simulink library "sm_wheel_loader_lib"  (R2025a)
settings: Solver=VariableStepAuto  StartTime=0.0  StopTime=10.0  RelTol=1e-3
undefined symbols (not defined in the file): AToTOrificeVector, BiPOrificeVector, boomHEArea, boomREArea, BToTOrificeVector, fluids, GRake, GToothL, GToothR, HMPST, HydFcnParams, logLoad, Position, PToAOrificeVector, PToBOrificeVector, RakeL, RakeR, testInput, Wheel_Loader, X, Y, Z
libraries: sm_lib x694, fl_lib x183, nesl_utility x74, SimscapeFluids_lib x62, sdl_lib x25, cvt_components_lib x25, simulink_extras x5, $bdroot x4, wheel_loader_contact_lib x4, ee_lib x2, SignalEditorBlockLib x1, batteryecm_lib x1
(part 3 of 26)

== system sm_wheel_loader_lib/CVT Power Split Hydromechanical/HRB ==
  str : Inport
  Constant : Constant  Value=HMPST.HRB.Pump.effVol
  Constant1 : Constant  Value=HMPST.HRB.Pump.effMech
  Custom Hydraulic Fluid : fl_lib/Isothermal Liquid/Utilities/Isothermal Liquid Properties (IL)  rho_L_atm=850 kg/m^3  bulk_modulus_model=foundation.enum.bulk_modulus_model.const  beta_gain=6  beta_L_atm=0.8e9 Pa  nu_atm=18e-6 m^2/s  p_atm=0.101325 MPa  p_min=1 Pa  properties_range_check=simscape.enum.assert.action.error  air_fraction=0.005  polytropic_index=1.0  rho_g_atm=1.225 kg/m^3  air_dissolution_model=simscape.enum.onoff.off  p_crit=3 MPa
      settings: LibrarySourceBlock=|
      | fl_lib/Hydraulic/Hydraulic Utilities/Custom Hydraulic
      | Fluid
  Gas-Charged Accumulator : SimscapeFluids_lib/Isothermal Liquid/Tanks & Accumulators/Gas-Charged Accumulator (IL)  capacity=HMPST.HRB.Accumulator.volTotal m^3  dead_volume=HMPST.HRB.Accumulator.volGasMin m^3  p_precharge=HMPST.HRB.Accumulator.pPrecharge MPa  k_sh=1.4  stiff_coeff=1e10 Pa/m^3  dynamic_compressibility=simscape.enum.onoff.off  liquid_volume_specify=on  liquid_volume_priority=High  liquid_volume=HMPST.HRB.Accumulator.volLiquidInit m^3  liquid_volume_nominal_specify=off  liquid_volume_nominal_value=1  liquid_volume_nominal_unit=m^3  liquid_mass_specify=off  liquid_mass_priority=None  liquid_mass=5 kg  liquid_mass_nominal_specify=off  liquid_mass_nominal_value=1  liquid_mass_nominal_unit=kg  p_I_specify=on  p_I_priority=None  p_I=HMPST.HRB.Accumulator.pLiquidInit Pa  p_I_nominal_specify=off  p_I_nominal_value=1  p_I_nominal_unit=Pa
      settings: InternalSimscapePortConfiguration="{\"Bottom\":[],\"Left\":[],\"Right\":[{\"id\":\"A\",\"label\":\"A\",\"type\":\"foundation.isothermal_liquid.isothermal_liquid\"}],\"Top\":[]}"
      settings: LibrarySourceBlock=|
      | sh_lib/Accumulators/Gas-Charged
      | Accumulator
  Maximum displacement : fl_lib/Physical Signals/Nonlinear Operators/PS Saturation  upper_limit=HMPST.HRB.Pump.dispMax m^3/rad  lower_limit=HMPST.HRB.Pump.dispMin m^3/rad  ZeroCross=true
  Mechanical Rotational Reference : fl_lib/Mechanical/Rotational Elements/Mechanical Rotational Reference
  Pressure Relief Valve : SimscapeFluids_lib/Isothermal Liquid/Valves & Orifices/Pressure Control Valves/Pressure Relief Valve (IL)  set_pressure_spec=foundation.enum.constant_controlled.constant  opening_spec=1  pressure_spec=fluids.isothermal_liquid.valves_orifices.enum.pressure_control_spec.dp  p_set_gauge=0.1 MPa  p_set_differential=HMPST.HRB.PRV.pDiffOpen bar  p_range=HMPST.HRB.PRV.pRange bar  area_max=HMPST.HRB.PRV.aMax m^2  area_leak=HMPST.HRB.PRV.aLeak m^2  p_diff_TLU=[30.15e5 : 15e3 : 31.35e5] Pa  p_gauge_TLU=[0.2 : 0.2 : 1.2] MPa  valve_area_TLU=[1 : 1 : 9] .* 1e-5 m^2  vol_flow_TLU=[1e-09, 3.6e-05, 8.9e-05, .00015, .00023, .00031] m^3/s  area=inf m^2  Cd=0.7  Re_c=12  smoothing_factor=0  pressure_recovery=false  opening_dynamics=1  tau=HMPST.HRB.PRV.tsOpen s
      settings: InternalSimscapePortConfiguration="{\"Bottom\":[],\"Left\":[{\"id\":\"A\",\"label\":\"A\",\"type\":\"foundation.isothermal_liquid.isothermal_liquid\"}],\"Right\":[{\"id\":\"B\",\"label\":\"B\",\"type\":\"foundation.isothermal_liquid.isothermal_liquid\"}],\"Top\":[]}"
      settings: LibrarySourceBlock=|
      | sh_lib/Valves/Pressure Control
      | Valves/Pressure Relief
      | Valve
  Reservoir : fl_lib/Isothermal Liquid/Elements/Reservoir (IL)  reservoir_type=foundation.enum.constant_controlled.constant  pressure_spec=foundation.enum.pressure_spec.atmospheric  reservoir_pressure=0.101325 MPa
      settings: LibrarySourceBlock=fl_lib/Hydraulic/Hydraulic Elements/Hydraulic Reference
  Simulink-PS Converter : nesl_utility/Simulink-PS Converter  PhysicalDomain=network_engine_domain  SubClassName=ps_input  LeftPortType=input  RightPortType=output  PseudoPeriodic=off  Frequencies=[]  NoiseDistribution=none  NoiseParameters=[]  Unit=1  AffineConversion=off  FilteringAndDerivatives=zero  SimscapeFilterOrder=1  InputFilterTimeConstant=0.001  UdotUserProvided=1
  Simulink-PS Converter1 : nesl_utility/Simulink-PS Converter  PhysicalDomain=network_engine_domain  SubClassName=ps_input  LeftPortType=input  RightPortType=output  PseudoPeriodic=off  Frequencies=[]  NoiseDistribution=none  NoiseParameters=[]  Unit=1  AffineConversion=off  FilteringAndDerivatives=zero  SimscapeFilterOrder=1  InputFilterTimeConstant=0.001  UdotUserProvided=1
  Simulink-PS Converter3 : nesl_utility/Simulink-PS Converter  PhysicalDomain=network_engine_domain  SubClassName=ps_input  LeftPortType=input  RightPortType=output  PseudoPeriodic=off  Frequencies=[]  NoiseDistribution=none  NoiseParameters=[]  Unit=m  AffineConversion=off  FilteringAndDerivatives=zero  SimscapeFilterOrder=1  InputFilterTimeConstant=0.001  UdotUserProvided=1
  Subsystem : Subsystem
  Transfer Fcn7 : TransferFcn  Numerator=HMPST.Ctrl.HRB.Num  Denominator=HMPST.Ctrl.HRB.Den
  Variable-Displacement Hydraulic Machine : SimscapeFluids_lib/Isothermal Liquid/Pumps & Motors/Variable-Displacement Motor (IL)  leakage_friction_spec=fluids.isothermal_liquid.pumps_motors.enum.pump_motor_loss_spec.input_efficiency  displacement_nominal=30 cm^3/rev  omega_nominal=1800 rpm  p_nominal=10 MPa  vol_eff_nominal=0.92  mech_eff_nominal=0.88  no_load_torque=0 N*m  p_diff_eff_TLU=[.1, 1, 2] MPa  omega_eff_TLU=[250, 500, 1000, 2000, 3000, 4000] rpm  displacement_eff_TLU=[-30, -19, 19, 30] cm^3/rev  vol_eff_TLU=repmat([.816, .908, .954, .977, .981, .984; .325, .663, .831, .916, .925, .946; .137, .568, .78, .892, .893, .91], 1, 1, 4)  mech_eff_TLU=repmat([.996, .996, .996, .996, .996, .996; .988, .989, .989, .989, .989, .99; .981, .981, .982, .982, .983, .984], 1, 1, 4)  p_diff_loss_TLU=[.1, 1, 2] MPa  omega_loss_TLU=[250, 500, 1000, 2000, 3000, 4000] rpm  displacement_loss_TLU=[-30, -19, 19, 30] cm^3/rev  vol_loss_TLU=repmat(1e-3 * [.023, .023, .023, .023, .0285, .032; .0844, .0842, .0845, .084, .1125, .108; .1079, .108, .11, .108, .1605, .18], 1, 1, 4) m^3/s  mech_loss_TLU=repmat([.002, .002, .002, .002, .002, .002; .0607, .0556, .0556, .0556, .0556, .0505; .1937, .1937, .1833, .1833, .1729, .1626], 1, 1, 4) N*m  vol_eff_min=1e-3  vol_eff_max=1  mech_eff_min=1e-3  mech_eff_max=1  pressure_threshold=1e-3 MPa  omega_threshold=100 rpm  displacement_threshold=0.1 cm^3/rev  supplied_range_check=simscape.enum.assert.action.none  motor_mode_check=simscape.enum.assert.action.none  pressure_check=simscape.enum.assert.action.none  p_min_valid=0.101325 MPa
      settings: InternalSimscapePortConfiguration="{\"Bottom\":[{\"id\":\"B\",\"label\":\"B\",\"type\":\"foundation.isothermal_liquid.isothermal_liquid\"}],\"Left\":[{\"id\":\"D\",\"label\":\"D\",\"type\":\"input\"},{\"id\":\"EV\",\"label\":\"EV\",\"type\":\"input\"},{\"id\":\"EM\",\"label\":\"EM\",\"type\":\"input\"}],\"Right\":[{\"id\":\"R\",\"label\":\"R\",\"type\":\"foundation.mechanical.rotational.rotational\"},{\"id\":\"C\",\"label\":\"C\",\"type\":\"foundation.mechanical.rotational.rotational\"}],\"Top\":[{\"id\":\"A\",\"label\":\"A\",\"type\":\"foundation.isothermal_liquid.isothermal_liquid\"}]}"
      settings: LibrarySourceBlock=|
      | sh_legacy_lib/Hydraulic Machines/Variable-Displacement
      | Hydraulic Machine
      | (External
      | Efficiencies)
  stroke2disp : fl_lib/Physical Signals/Functions/PS Gain  gain=HMPST.HRB.Pump.stroke2disp m^2/rad
  R : PMIOPort  Side=Right
  p : Outport
  wires:
  Transfer Fcn7/1 -> Simulink-PS Converter3/1  "HRB"
  str/1 -> Transfer Fcn7/1
  Constant/1 -> Simulink-PS Converter/1
  Constant1/1 -> Simulink-PS Converter1/1
  Subsystem/1(p) -> p/1  "P_acc (MPa)"
  connections:
  Subsystem/LConn1 -- Pressure Relief Valve/LConn1 -- Variable-Displacement Hydraulic Machine/RConn3 -- Gas-Charged Accumulator/RConn1
  stroke2disp/RConn1 -- Maximum displacement/LConn1
  R/RConn1 -- Variable-Displacement Hydraulic Machine/RConn1
  Simulink-PS Converter3/RConn1 -- stroke2disp/LConn1
  Maximum displacement/RConn1 -- Variable-Displacement Hydraulic Machine/LConn1
  Pressure Relief Valve/RConn1 -- Reservoir/LConn1 -- Variable-Displacement Hydraulic Machine/LConn4 -- Custom Hydraulic Fluid/RConn1
  Mechanical Rotational Reference/LConn1 -- Variable-Displacement Hydraulic Machine/RConn2
  Variable-Displacement Hydraulic Machine/LConn3 -- Simulink-PS Converter1/RConn1
  Variable-Displacement Hydraulic Machine/LConn2 -- Simulink-PS Converter/RConn1

== system sm_wheel_loader_lib/CVT Power Split Hydromechanical/Hydrostatic ==
  Ctrl : Inport
  CV Charge Pump : fl_lib/Isothermal Liquid/Elements/Constant Volume Chamber (IL)  volume=1e-4 m^3  p_I_specify=off  p_I_priority=High  p_I=0.101325 MPa  p_I_nominal_specify=off  p_I_nominal_value=1  p_I_nominal_unit=MPa
      settings: InternalSimscapePortConfiguration="{\"Bottom\":[],\"Left\":[{\"id\":\"A\",\"label\":\"A\",\"type\":\"foundation.isothermal_liquid.isothermal_liquid\"}],\"Right\":[],\"Top\":[]}"
  CV Motor A : fl_lib/Isothermal Liquid/Elements/Constant Volume Chamber (IL)  volume=1e-4 m^3  p_I_specify=off  p_I_priority=High  p_I=0.101325 MPa  p_I_nominal_specify=off  p_I_nominal_value=1  p_I_nominal_unit=MPa
      settings: InternalSimscapePortConfiguration="{\"Bottom\":[],\"Left\":[{\"id\":\"A\",\"label\":\"A\",\"type\":\"foundation.isothermal_liquid.isothermal_liquid\"}],\"Right\":[],\"Top\":[]}"
  CV Motor B : fl_lib/Isothermal Liquid/Elements/Constant Volume Chamber (IL)  volume=1e-4 m^3  p_I_specify=off  p_I_priority=High  p_I=0.101325 MPa  p_I_nominal_specify=off  p_I_nominal_value=1  p_I_nominal_unit=MPa
      settings: InternalSimscapePortConfiguration="{\"Bottom\":[],\"Left\":[{\"id\":\"A\",\"label\":\"A\",\"type\":\"foundation.isothermal_liquid.isothermal_liquid\"}],\"Right\":[],\"Top\":[]}"
  CV Pump A : fl_lib/Isothermal Liquid/Elements/Constant Volume Chamber (IL)  volume=1e-4 m^3  p_I_specify=off  p_I_priority=High  p_I=0.101325 MPa  p_I_nominal_specify=off  p_I_nominal_value=1  p_I_nominal_unit=MPa
      settings: InternalSimscapePortConfiguration="{\"Bottom\":[],\"Left\":[{\"id\":\"A\",\"label\":\"A\",\"type\":\"foundation.isothermal_liquid.isothermal_liquid\"}],\"Right\":[],\"Top\":[]}"
  CV Pump B : fl_lib/Isothermal Liquid/Elements/Constant Volume Chamber (IL)  volume=1e-4 m^3  p_I_specify=off  p_I_priority=High  p_I=0.101325 MPa  p_I_nominal_specify=off  p_I_nominal_value=1  p_I_nominal_unit=MPa
      settings: InternalSimscapePortConfiguration="{\"Bottom\":[],\"Left\":[{\"id\":\"A\",\"label\":\"A\",\"type\":\"foundation.isothermal_liquid.isothermal_liquid\"}],\"Right\":[],\"Top\":[]}"
  Charge Pump : Subsystem  Tag=PublishSubsystem  mask{chgPumpNomDisp=chgPumpNomDisp, chgPumpNomSpd=chgPumpNomSpd, chgPumpNomPressGain=chgPumpNomPressGain, chgPumpNomVolEff=chgPumpNomVolEff, chgPumpNomMechEff=chgPumpNomMechEff, chgPumpChkvPdiff=chgPumpChkvPdiff, chgPumpChkvPrange=chgPumpChkvPrange, chgPumpChkvAmax=chgPumpChkvAmax, chgPumpChkvAleak=chgPumpChkvAleak}
      mask prompts: chgPumpNomDisp "Displacement (cm^3/rev)"; chgPumpNomSpd "Nominal Angular Velocity (rpm)"; chgPumpNomPressGain "Nominal pressure gain (MPa)"; chgPumpNomVolEff "Nominal Volumetric Efficiency (0-1)"; chgPumpNomMechEff "Nominal Mechanical Efficiency (0-1)"; chgPumpChkvPdiff "Set pressure differential (MPa)"; chgPumpChkvPrange "Pressure regulation range (MPa)"; chgPumpChkvAmax "Maximum opening area (m^2)"; chgPumpChkvAleak "Leakage area (m^2)"
      mask TypeOptions chgPumpNomDisp: Pump/displacement
      mask TypeOptions chgPumpNomSpd: Pump/omega_nominal
      mask TypeOptions chgPumpNomPressGain: Pump/p_nominal
      mask TypeOptions chgPumpNomVolEff: Pump/vol_eff_nominal
      mask TypeOptions chgPumpNomMechEff: Pump/mech_eff_nominal
      mask TypeOptions chgPumpChkvPdiff:
      | Pressure
      | Relief
      | Valve/p_set_differential
      mask TypeOptions chgPumpChkvPrange:
      | Pressure
      | Relief
      | Valve/p_range
      mask TypeOptions chgPumpChkvAmax:
      | Pressure
      | Relief
      | Valve/area_max
      mask TypeOptions chgPumpChkvAleak:
      | Pressure
      | Relief
      | Valve/area_leak
      mask DialogControl grp_chg_pump Prompt: Pump
      mask DialogControl grp_chg_pump_prv Prompt: Pressure Relief Valve
      mask Display:
      | % Circle
      | color('green')
      | plot(2*cos(linspace(0, 2*pi, 100)), 2*sin(linspace(0, 2*pi, 100)))
      | % Triangle
      | patch([1 0.4 0.4]*2, [0,-0.4,0.4]*2,[45 48 173]/255)
      | % Boundary
      | color('white')
      | plot(-2, -2)
      | plot(2, 2)
  Check Valve A : SimscapeFluids_lib/Isothermal Liquid/Valves & Orifices/Directional Control Valves/Check Valve (IL)  opening_spec=2*(fluids.isothermal_liquid.valves_orifices.enum.PressureOpeningSpec.Linear)-1  pressure_control_spec=fluids.isothermal_liquid.valves_orifices.enum.pressure_control_spec.dp  p_crack_differential=p_crack_differential MPa  p_crack_gauge=0.1 MPa  press_max_differential=press_max_differential MPa  press_max_gauge=0.2 MPa  area_max=chkv_area_max m^2  area_leak=chkv_area_leak m^2  p_diff_TLU=[0.01 : 0.01 : 0.1] MPa  valve_area_TLU=[1e-10, 1e-05, 2e-05, 3e-05, 4e-05, 5e-05, 6e-05, 7.5e-05, 8.5e-05, .0001] m^2  vol_flow_TLU=[.000358, .045, .11, .191, .284, .39, .505, .63, .764, .905] .* 1e-3 m^3/s  area=inf m^2  Cd=0.64  Re_c=150  smoothing_factor=0.01  pressure_recovery=simscape.enum.onoff.off  opening_dynamics=simscape.enum.onoff.off  tau=0.1 s
      settings: InternalSimscapePortConfiguration="{\"Bottom\":[],\"Left\":[{\"id\":\"A\",\"label\":\"A\",\"type\":\"foundation.isothermal_liquid.isothermal_liquid\"}],\"Right\":[{\"id\":\"B\",\"label\":\"B\",\"type\":\"foundation.isothermal_liquid.isothermal_liquid\"}],\"Top\":[]}"
  Check Valve B : SimscapeFluids_lib/Isothermal Liquid/Valves & Orifices/Directional Control Valves/Check Valve (IL)  opening_spec=2*(fluids.isothermal_liquid.valves_orifices.enum.PressureOpeningSpec.Linear)-1  pressure_control_spec=fluids.isothermal_liquid.valves_orifices.enum.pressure_control_spec.dp  p_crack_differential=p_crack_differential MPa  p_crack_gauge=0.1 MPa  press_max_differential=press_max_differential MPa  press_max_gauge=0.2 MPa  area_max=chkv_area_max m^2  area_leak=chkv_area_leak m^2  p_diff_TLU=[0.01 : 0.01 : 0.1] MPa  valve_area_TLU=[1e-10, 1e-05, 2e-05, 3e-05, 4e-05, 5e-05, 6e-05, 7.5e-05, 8.5e-05, .0001] m^2  vol_flow_TLU=[.000358, .045, .11, .191, .284, .39, .505, .63, .764, .905] .* 1e-3 m^3/s  area=inf m^2  Cd=0.64  Re_c=150  smoothing_factor=0.01  pressure_recovery=simscape.enum.onoff.off  opening_dynamics=simscape.enum.onoff.off  tau=0.1 s
      settings: InternalSimscapePortConfiguration="{\"Bottom\":[],\"Left\":[{\"id\":\"A\",\"label\":\"A\",\"type\":\"foundation.isothermal_liquid.isothermal_liquid\"}],\"Right\":[{\"id\":\"B\",\"label\":\"B\",\"type\":\"foundation.isothermal_liquid.isothermal_liquid\"}],\"Top\":[]}"
  Gain1 : Gain  Gain=pumpNomDisp
  Gain2 : Gain  Gain=-1
  Mechanical Rotational Reference : fl_lib/Mechanical/Rotational Elements/Mechanical Rotational Reference
  Mechanical Rotational Reference1 : fl_lib/Mechanical/Rotational Elements/Mechanical Rotational Reference
  Motor : SimscapeFluids_lib/Isothermal Liquid/Pumps & Motors/Fixed-Displacement Motor (IL)  leakage_friction_spec=fluids.isothermal_liquid.pumps_motors.enum.MotorLossSpec.Analytical  displacement=motorNomDisp cm^3/rev  omega_nominal=motorNomSpd rpm  p_nominal=motorNomPressDrop MPa  vol_eff_nominal=motorNomVolEff  mech_eff_nominal=motorNomMechEff  no_load_torque=0 N*m  p_diff_eff_TLU=[.1, 1, 2] MPa  omega_eff_TLU=[25, 50, 100, 200, 300, 400] rad/s  vol_eff_TLU=[.816, .908, .954, .977, .981, .984; .325, .663, .831, .916, .925, .946; .137, .568, .78, .892, .893, .91]  mech_eff_TLU=[.996, .996, .996, .996, .996, .996; .988, .989, .989, .989, .989, .99; .981, .981, .982, .982, .983, .984]  p_diff_loss_TLU=[.1, 1, 2] MPa  omega_loss_TLU=[25, 50, 100, 200, 300, 400] rad/s  vol_loss_TLU=[.023, .023, .023, .023, .0285, .032; .0844, .0842, .0845, .084, .1125, .108; .1079, .108, .11, .108, .1605, .18] * 1e-3 m^3/s  mech_loss_TLU=[.002, .002, .002, .002, .002, .002; .0607, .0556, .0556, .0556, .0556, .0505; .1937, .1937, .1833, .1833, .1729, .1626] N*m  q_shaft_TLU=[.125, .25, .5, 1, 1.5, 2] * 1e-3 m^3/s  p_diff_shaft_TLU=[.1, 1, 2] MPa  torque_shaft_TLU=[.47, 4.72, 9.35; .47, 4.7, 9.36; .47, 4.7, 9.4; .47, 4.7, 9.41; .47, 4.7, 9.46; .47, 4.68, 9.5] N*m  omega_shaft_TLU=[205, 80, 35; 455, 330, 285; 955, 831, 780; 1950, 1830, 1780; 2940, 2775, 2680; 3940, 3780, 3640] rpm  vol_eff_min=1e-3  vol_eff_max=1  mech_eff_min=1e-3  mech_eff_max=1  pressure_threshold=1e-3 MPa  omega_threshold=10 rad/s  supplied_range_check=simscape.enum.assert.action.none  motor_mode_check=simscape.enum.assert.action.none  pressure_check=simscape.enum.assert.action.none  p_min_valid=0.101325 MPa
      settings: InternalSimscapePortConfiguration="{\"Bottom\":[{\"id\":\"B\",\"label\":\"B\",\"type\":\"foundation.isothermal_liquid.isothermal_liquid\"}],\"Left\":[],\"Right\":[{\"id\":\"R\",\"label\":\"R\",\"type\":\"foundation.mechanical.rotational.rotational\"},{\"id\":\"C\",\"label\":\"C\",\"type\":\"foundation.mechanical.rotational.rotational\"}],\"Top\":[{\"id\":\"A\",\"label\":\"A\",\"type\":\"foundation.isothermal_liquid.isothermal_liquid\"}]}"
  Motor Leakage : Subsystem  Tag=PublishSubsystem
  "Pipe A " : fl_lib/Isothermal Liquid/Elements/Pipe (IL)  length=pipeLen m  area=pipeAreaGeo m^2  Dh=pipeAreaHydr m  length_add=4 m  roughness=15e-6 m  Re_lam=2000  Re_tur=4000  shape_factor=64  dynamic_compressibility=simscape.enum.onoff.on  inertia=simscape.enum.onoff.off  p0=0.101325 MPa  mdot0=0 kg/s
      settings: InternalSimscapePortConfiguration="{\"Bottom\":[],\"Left\":[{\"id\":\"A\",\"label\":\"A\",\"type\":\"foundation.isothermal_liquid.isothermal_liquid\"}],\"Right\":[{\"id\":\"B\",\"label\":\"B\",\"type\":\"foundation.isothermal_liquid.isothermal_liquid\"}],\"Top\":[]}"
  Pipe B : fl_lib/Isothermal Liquid/Elements/Pipe (IL)  length=pipeLen m  area=pipeAreaGeo m^2  Dh=pipeAreaHydr m  length_add=4 m  roughness=15e-6 m  Re_lam=2000  Re_tur=4000  shape_factor=64  dynamic_compressibility=simscape.enum.onoff.on  inertia=simscape.enum.onoff.off  p0=0.101325 MPa  mdot0=0 kg/s
      settings: InternalSimscapePortConfiguration="{\"Bottom\":[],\"Left\":[{\"id\":\"A\",\"label\":\"A\",\"type\":\"foundation.isothermal_liquid.isothermal_liquid\"}],\"Right\":[{\"id\":\"B\",\"label\":\"B\",\"type\":\"foundation.isothermal_liquid.isothermal_liquid\"}],\"Top\":[]}"
  Pressure Relief Valve A : SimscapeFluids_lib/Isothermal Liquid/Valves & Orifices/Pressure Control Valves/Pressure Relief Valve (IL)  set_pressure_spec=foundation.enum.constant_controlled.constant  opening_spec=fluids.isothermal_liquid.valves_orifices.enum.opening_spec.linear  pressure_spec=fluids.isothermal_liquid.valves_orifices.enum.pressure_control_spec.dp  p_set_gauge=0.1 MPa  p_set_differential=p_set_differential MPa  p_range=p_range MPa  area_max=prv_area_max m^2  area_leak=prv_area_leak m^2  p_diff_TLU=[0.2 : 0.2 : 1.2] MPa  p_gauge_TLU=[0.2 : 0.2 : 1.2] MPa  valve_area_TLU=[1e-10, 2e-06, 4e-06, 6e-06, 8e-06, 1e-05] m^2  vol_flow_TLU=[1e-09, 3.6e-05, 8.9e-05, .00015, .00023, .00031] m^3/s  area=inf m^2  Cd=0.64  Re_c=150  smoothing_factor=0.01  pressure_recovery=simscape.enum.onoff.off  opening_dynamics=simscape.enum.onoff.off  tau=0.1 s
      settings: InternalSimscapePortConfiguration="{\"Bottom\":[],\"Left\":[{\"id\":\"A\",\"label\":\"A\",\"type\":\"foundation.isothermal_liquid.isothermal_liquid\"}],\"Right\":[{\"id\":\"B\",\"label\":\"B\",\"type\":\"foundation.isothermal_liquid.isothermal_liquid\"}],\"Top\":[]}"
  Pressure Relief Valve B : SimscapeFluids_lib/Isothermal Liquid/Valves & Orifices/Pressure Control Valves/Pressure Relief Valve (IL)  set_pressure_spec=foundation.enum.constant_controlled.constant  opening_spec=fluids.isothermal_liquid.valves_orifices.enum.opening_spec.linear  pressure_spec=fluids.isothermal_liquid.valves_orifices.enum.pressure_control_spec.dp  p_set_gauge=0.1 MPa  p_set_differential=p_set_differential MPa  p_range=p_range MPa  area_max=prv_area_max m^2  area_leak=prv_area_leak m^2  p_diff_TLU=[0.2 : 0.2 : 1.2] MPa  p_gauge_TLU=[0.2 : 0.2 : 1.2] MPa  valve_area_TLU=[1e-10, 2e-06, 4e-06, 6e-06, 8e-06, 1e-05] m^2  vol_flow_TLU=[1e-09, 3.6e-05, 8.9e-05, .00015, .00023, .00031] m^3/s  area=inf m^2  Cd=0.64  Re_c=150  smoothing_factor=0.01  pressure_recovery=simscape.enum.onoff.off  opening_dynamics=simscape.enum.onoff.off  tau=0.1 s
      settings: InternalSimscapePortConfiguration="{\"Bottom\":[],\"Left\":[{\"id\":\"A\",\"label\":\"A\",\"type\":\"foundation.isothermal_liquid.isothermal_liquid\"}],\"Right\":[{\"id\":\"B\",\"label\":\"B\",\"type\":\"foundation.isothermal_liquid.isothermal_liquid\"}],\"Top\":[]}"
  Pump : SimscapeFluids_lib/Isothermal Liquid/Pumps & Motors/Variable-Displacement Pump (IL)  leakage_friction_spec=fluids.isothermal_liquid.pumps_motors.enum.pump_motor_loss_spec.analytical  displacement_nominal=pumpNomDisp cm^3/rev  omega_nominal=pumpNomSpd rpm  p_nominal=pumpNomPressGain MPa  vol_eff_nominal=pumpNomVolEff  mech_eff_nominal=pumpNomMechEff  no_load_torque=0 N*m  p_diff_eff_TLU=[.1, 1, 2] MPa  omega_eff_TLU=[25, 50, 100, 200, 300, 400] rad/s  displacement_eff_TLU=[-30, -19, 19, 30] cm^3/rev  vol_eff_TLU=repmat([.816, .908, .954, .977, .981, .984; .325, .663, .831, .916, .925, .946; .137, .568, .78, .892, .893, .91], 1, 1, 4)  mech_eff_TLU=repmat([.996, .996, .996, .996, .996, .996; .988, .989, .989, .989, .989, .99; .981, .981, .982, .982, .983, .984], 1, 1, 4)  p_diff_loss_TLU=[.1, 1, 2] MPa  omega_loss_TLU=[25, 50, 100, 200, 300, 400] rad/s  displacement_loss_TLU=[-30, -19, 19, 30] cm^3/rev  vol_loss_TLU=repmat([.023, .023, .023, .023, .0285, .032; .0844, .0842, .0845, .084, .1125, .108; .1079, .108, .11, .108, .1605, .18] * 1e-3, 1, 1, 4) m^3/s  mech_loss_TLU=repmat([.002, .002, .002, .002, .002, .002; .0607, .0556, .0556, .0556, .0556, .0505; .1937, .1937, .1833, .1833, .1729, .1626], 1, 1, 4) N*m  vol_eff_min=1e-3  vol_eff_max=1  mech_eff_min=1e-3  mech_eff_max=1  pressure_threshold=1e-3 MPa  omega_threshold=10 rad/s  displacement_threshold=0.1 cm^3/rev  supplied_range_check=simscape.enum.assert.action.none  pump_mode_check=simscape.enum.assert.action.none  pressure_check=simscape.enum.assert.action.none  p_min_valid=0.101325 MPa
      settings: InternalSimscapePortConfiguration="{\"Bottom\":[{\"id\":\"A\",\"label\":\"A\",\"type\":\"foundation.isothermal_liquid.isothermal_liquid\"}],\"Left\":[{\"id\":\"D\",\"label\":\"D\",\"type\":\"input\"}],\"Right\":[{\"id\":\"R\",\"label\":\"R\",\"type\":\"foundation.mechanical.rotational.rotational\"},{\"id\":\"C\",\"label\":\"C\",\"type\":\"foundation.mechanical.rotational.rotational\"}],\"Top\":[{\"id\":\"B\",\"label\":\"B\",\"type\":\"foundation.isothermal_liquid.isothermal_liquid\"}]}"
  Pump Leakage : Subsystem  Tag=PublishSubsystem
  Simulink-PS Converter1 : nesl_utility/Simulink-PS Converter  PhysicalDomain=network_engine_domain  SubClassName=ps_input  LeftPortType=input  RightPortType=output  PseudoPeriodic=off  Frequencies=[]  NoiseDistribution=none  NoiseParameters=[]  Unit=cm^3/rev  AffineConversion=off  FilteringAndDerivatives=provide  SimscapeFilterOrder=1  InputFilterTimeConstant=0.001  UdotUserProvided=0
  Transmission Fluid Properties : fl_lib/Isothermal Liquid/Utilities/Isothermal Liquid Properties (IL)  rho_L_atm=850 kg/m^3  bulk_modulus_model=foundation.enum.bulk_modulus_model.const  beta_gain=6  beta_L_atm=1.4 GPa  nu_atm=18.8 cSt  p_atm=0.101325 MPa  p_min=0.1 Pa  properties_range_check=simscape.enum.assert.action.error  air_fraction=0.005  polytropic_index=1.0  rho_g_atm=1.225 kg/m^3  air_dissolution_model=simscape.enum.onoff.off  p_crit=3 MPa
  In : PMIOPort  Side=Left
  Out : PMIOPort  Port=2  Side=Right
  wires:
  Ctrl/1 -> Gain2/1
  Gain1/1 -> Simulink-PS Converter1/1
  Gain2/1 -> Gain1/1
  connections:
  In/RConn1 -- Charge Pump/LConn1 -- Pump/RConn1
  Motor/RConn1 -- Out/RConn1
  Mechanical Rotational Reference1/LConn1 -- Pump/RConn2
  Pressure Relief Valve A/LConn1 -- Pressure Relief Valve B/RConn1 -- Motor Leakage/LConn1 -- CV Motor A/LConn1 -- Motor/LConn1 -- "Pipe A "/RConn1
  Motor/RConn2 -- Mechanical Rotational Reference/LConn1
  Check Valve B/LConn1 -- Check Valve A/LConn1 -- Charge Pump/RConn1 -- CV Charge Pump/LConn1
  Check Valve A/RConn1 -- Pump Leakage/LConn1 -- Transmission Fluid Properties/RConn1 -- CV Pump B/LConn1 -- Pump/LConn2 -- "Pipe A "/LConn1
  Check Valve B/RConn1 -- Pump Leakage/LConn2 -- CV Pump A/LConn1 -- Pump/RConn3 -- Pipe B/LConn1
  Pressure Relief Valve A/RConn1 -- Pressure Relief Valve B/LConn1 -- Motor Leakage/LConn2 -- CV Motor B/LConn1 -- Motor/RConn3 -- Pipe B/RConn1
  Simulink-PS Converter1/RConn1 -- Pump/LConn1

== system sm_wheel_loader_lib/CVT Power Split Hydromechanical/Sensor P1s ==
  MRRef : fl_lib/Mechanical/Rotational Elements/Mechanical Rotational Reference
  Motion Sensor : fl_lib/Mechanical/Mechanical Sensors/Ideal Rotational Motion Sensor  reference=foundation.enum.MeasurementReference.difference  acceleration_port=false  velocity_port=true  position_port=false  wrap_angle=false  offset=0 rad
      settings: InternalSimscapePortConfiguration="{\"Bottom\":[],\"Left\":[{\"id\":\"R\",\"label\":\"R\",\"type\":\"foundation.mechanical.rotational.rotational\"}],\"Right\":[{\"id\":\"C\",\"label\":\"C\",\"type\":\"foundation.mechanical.rotational.rotational\"},{\"id\":\"W\",\"label\":\"W\",\"type\":\"output\"}],\"Top\":[]}"
  PS-Simulink Converter : nesl_utility/PS-Simulink Converter  PhysicalDomain=network_engine_domain  SubClassName=ps_output  LeftPortType=input  RightPortType=output  PseudoPeriodic=off  Frequencies=[]  VectorFormat=inherit  Unit=rpm  AffineConversion=off
  R : PMIOPort  Side=Left
  w : Outport
  wires:
  PS-Simulink Converter/1 -> w/1
  connections:
  R/RConn1 -- Motion Sensor/LConn1
  MRRef/LConn1 -- Motion Sensor/RConn1
  PS-Simulink Converter/LConn1 -- Motion Sensor/RConn2

== system sm_wheel_loader_lib/CVT Power Split Hydromechanical/Sensor wG2 ==
  MRRef : fl_lib/Mechanical/Rotational Elements/Mechanical Rotational Reference
  Motion Sensor : fl_lib/Mechanical/Mechanical Sensors/Ideal Rotational Motion Sensor  reference=foundation.enum.MeasurementReference.difference  acceleration_port=false  velocity_port=true  position_port=false  wrap_angle=false  offset=0 rad
      settings: InternalSimscapePortConfiguration="{\"Bottom\":[],\"Left\":[{\"id\":\"R\",\"label\":\"R\",\"type\":\"foundation.mechanical.rotational.rotational\"}],\"Right\":[{\"id\":\"C\",\"label\":\"C\",\"type\":\"foundation.mechanical.rotational.rotational\"},{\"id\":\"W\",\"label\":\"W\",\"type\":\"output\"}],\"Top\":[]}"
  PS-Simulink Converter : nesl_utility/PS-Simulink Converter  PhysicalDomain=network_engine_domain  SubClassName=ps_output  LeftPortType=input  RightPortType=output  PseudoPeriodic=off  Frequencies=[]  VectorFormat=inherit  Unit=rpm  AffineConversion=off
  R : PMIOPort  Side=Left
  w : Outport
  wires:
  PS-Simulink Converter/1 -> w/1
  connections:
  R/RConn1 -- Motion Sensor/LConn1
  MRRef/LConn1 -- Motion Sensor/RConn1
  PS-Simulink Converter/LConn1 -- Motion Sensor/RConn2

== system sm_wheel_loader_lib/CVT Power Split Hydromechanical/Sensor wG3 ==
  MRRef : fl_lib/Mechanical/Rotational Elements/Mechanical Rotational Reference
  Motion Sensor : fl_lib/Mechanical/Mechanical Sensors/Ideal Rotational Motion Sensor  reference=foundation.enum.MeasurementReference.difference  acceleration_port=false  velocity_port=true  position_port=false  wrap_angle=false  offset=0 rad
      settings: InternalSimscapePortConfiguration="{\"Bottom\":[],\"Left\":[{\"id\":\"R\",\"label\":\"R\",\"type\":\"foundation.mechanical.rotational.rotational\"}],\"Right\":[{\"id\":\"C\",\"label\":\"C\",\"type\":\"foundation.mechanical.rotational.rotational\"},{\"id\":\"W\",\"label\":\"W\",\"type\":\"output\"}],\"Top\":[]}"
  PS-Simulink Converter : nesl_utility/PS-Simulink Converter  PhysicalDomain=network_engine_domain  SubClassName=ps_output  LeftPortType=input  RightPortType=output  PseudoPeriodic=off  Frequencies=[]  VectorFormat=inherit  Unit=rpm  AffineConversion=off
  R : PMIOPort  Side=Left
  w : Outport
  wires:
  PS-Simulink Converter/1 -> w/1
  connections:
  PS-Simulink Converter/LConn1 -- Motion Sensor/RConn2
  MRRef/LConn1 -- Motion Sensor/RConn1
  R/RConn1 -- Motion Sensor/LConn1

== system sm_wheel_loader_lib/CVT Power Split Hydromechanical/Sensor wG4 ==
  MRRef : fl_lib/Mechanical/Rotational Elements/Mechanical Rotational Reference
  Motion Sensor : fl_lib/Mechanical/Mechanical Sensors/Ideal Rotational Motion Sensor  reference=foundation.enum.MeasurementReference.difference  acceleration_port=false  velocity_port=true  position_port=false  wrap_angle=false  offset=0 rad
      settings: InternalSimscapePortConfiguration="{\"Bottom\":[],\"Left\":[{\"id\":\"R\",\"label\":\"R\",\"type\":\"foundation.mechanical.rotational.rotational\"}],\"Right\":[{\"id\":\"C\",\"label\":\"C\",\"type\":\"foundation.mechanical.rotational.rotational\"},{\"id\":\"W\",\"label\":\"W\",\"type\":\"output\"}],\"Top\":[]}"
  PS-Simulink Converter : nesl_utility/PS-Simulink Converter  PhysicalDomain=network_engine_domain  SubClassName=ps_output  LeftPortType=input  RightPortType=output  PseudoPeriodic=off  Frequencies=[]  VectorFormat=inherit  Unit=rpm  AffineConversion=off
  R : PMIOPort  Side=Left
  w : Outport
  wires:
  PS-Simulink Converter/1 -> w/1
  connections:
  PS-Simulink Converter/LConn1 -- Motion Sensor/RConn2
  MRRef/LConn1 -- Motion Sensor/RConn1
  R/RConn1 -- Motion Sensor/LConn1

== system sm_wheel_loader_lib/CVT Power Split Hydromechanical/Sensor wIn ==
  MRRef : fl_lib/Mechanical/Rotational Elements/Mechanical Rotational Reference
  Motion Sensor : fl_lib/Mechanical/Mechanical Sensors/Ideal Rotational Motion Sensor  reference=foundation.enum.MeasurementReference.difference  acceleration_port=false  velocity_port=true  position_port=false  wrap_angle=false  offset=0 rad
      settings: InternalSimscapePortConfiguration="{\"Bottom\":[],\"Left\":[{\"id\":\"R\",\"label\":\"R\",\"type\":\"foundation.mechanical.rotational.rotational\"}],\"Right\":[{\"id\":\"C\",\"label\":\"C\",\"type\":\"foundation.mechanical.rotational.rotational\"},{\"id\":\"W\",\"label\":\"W\",\"type\":\"output\"}],\"Top\":[]}"
  PS-Simulink Converter : nesl_utility/PS-Simulink Converter  PhysicalDomain=network_engine_domain  SubClassName=ps_output  LeftPortType=input  RightPortType=output  PseudoPeriodic=off  Frequencies=[]  VectorFormat=inherit  Unit=rpm  AffineConversion=off
  R : PMIOPort  Side=Left
  w : Outport
  wires:
  PS-Simulink Converter/1 -> w/1
  connections:
  PS-Simulink Converter/LConn1 -- Motion Sensor/RConn2
  MRRef/LConn1 -- Motion Sensor/RConn1
  R/RConn1 -- Motion Sensor/LConn1

== system sm_wheel_loader_lib/CVT Power Split Hydromechanical/Sensor wOut ==
  MRRef : fl_lib/Mechanical/Rotational Elements/Mechanical Rotational Reference
  Motion Sensor : fl_lib/Mechanical/Mechanical Sensors/Ideal Rotational Motion Sensor  reference=foundation.enum.MeasurementReference.difference  acceleration_port=false  velocity_port=true  position_port=false  wrap_angle=false  offset=0 rad
      settings: InternalSimscapePortConfiguration="{\"Bottom\":[],\"Left\":[{\"id\":\"R\",\"label\":\"R\",\"type\":\"foundation.mechanical.rotational.rotational\"}],\"Right\":[{\"id\":\"C\",\"label\":\"C\",\"type\":\"foundation.mechanical.rotational.rotational\"},{\"id\":\"W\",\"label\":\"W\",\"type\":\"output\"}],\"Top\":[]}"
  PS-Simulink Converter : nesl_utility/PS-Simulink Converter  PhysicalDomain=network_engine_domain  SubClassName=ps_output  LeftPortType=input  RightPortType=output  PseudoPeriodic=off  Frequencies=[]  VectorFormat=inherit  Unit=rpm  AffineConversion=off
  R : PMIOPort  Side=Left
  w : Outport
  wires:
  PS-Simulink Converter/1 -> w/1
  connections:
  R/RConn1 -- Motion Sensor/LConn1
  MRRef/LConn1 -- Motion Sensor/RConn1
  PS-Simulink Converter/LConn1 -- Motion Sensor/RConn2

== system sm_wheel_loader_lib/CVT Power Split Hydromechanical/Sensor wP1c ==
  MRRef : fl_lib/Mechanical/Rotational Elements/Mechanical Rotational Reference
  Motion Sensor : fl_lib/Mechanical/Mechanical Sensors/Ideal Rotational Motion Sensor  reference=foundation.enum.MeasurementReference.difference  acceleration_port=false  velocity_port=true  position_port=false  wrap_angle=false  offset=0 rad
      settings: InternalSimscapePortConfiguration="{\"Bottom\":[],\"Left\":[{\"id\":\"R\",\"label\":\"R\",\"type\":\"foundation.mechanical.rotational.rotational\"}],\"Right\":[{\"id\":\"C\",\"label\":\"C\",\"type\":\"foundation.mechanical.rotational.rotational\"},{\"id\":\"W\",\"label\":\"W\",\"type\":\"output\"}],\"Top\":[]}"
  PS-Simulink Converter : nesl_utility/PS-Simulink Converter  PhysicalDomain=network_engine_domain  SubClassName=ps_output  LeftPortType=input  RightPortType=output  PseudoPeriodic=off  Frequencies=[]  VectorFormat=inherit  Unit=rpm  AffineConversion=off
  R : PMIOPort  Side=Left
  w : Outport
  wires:
  PS-Simulink Converter/1 -> w/1
  connections:
  R/RConn1 -- Motion Sensor/LConn1
  MRRef/LConn1 -- Motion Sensor/RConn1
  PS-Simulink Converter/LConn1 -- Motion Sensor/RConn2

== system sm_wheel_loader_lib/CVT Power Split Hydromechanical/Sensor wP2s ==
  MRRef : fl_lib/Mechanical/Rotational Elements/Mechanical Rotational Reference
  Motion Sensor : fl_lib/Mechanical/Mechanical Sensors/Ideal Rotational Motion Sensor  reference=foundation.enum.MeasurementReference.difference  acceleration_port=false  velocity_port=true  position_port=false  wrap_angle=false  offset=0 rad
      settings: InternalSimscapePortConfiguration="{\"Bottom\":[],\"Left\":[{\"id\":\"R\",\"label\":\"R\",\"type\":\"foundation.mechanical.rotational.rotational\"}],\"Right\":[{\"id\":\"C\",\"label\":\"C\",\"type\":\"foundation.mechanical.rotational.rotational\"},{\"id\":\"W\",\"label\":\"W\",\"type\":\"output\"}],\"Top\":[]}"
  PS-Simulink Converter : nesl_utility/PS-Simulink Converter  PhysicalDomain=network_engine_domain  SubClassName=ps_output  LeftPortType=input  RightPortType=output  PseudoPeriodic=off  Frequencies=[]  VectorFormat=inherit  Unit=rpm  AffineConversion=off
  R : PMIOPort  Side=Left
  w : Outport
  wires:
  PS-Simulink Converter/1 -> w/1
  connections:
  PS-Simulink Converter/LConn1 -- Motion Sensor/RConn2
  MRRef/LConn1 -- Motion Sensor/RConn1
  R/RConn1 -- Motion Sensor/LConn1

== system sm_wheel_loader_lib/CVT Power Split Hydromechanical/Sensor wP3r ==
  MRRef : fl_lib/Mechanical/Rotational Elements/Mechanical Rotational Reference
  Motion Sensor : fl_lib/Mechanical/Mechanical Sensors/Ideal Rotational Motion Sensor  reference=foundation.enum.MeasurementReference.difference  acceleration_port=false  velocity_port=true  position_port=false  wrap_angle=false  offset=0 rad
      settings: InternalSimscapePortConfiguration="{\"Bottom\":[],\"Left\":[{\"id\":\"R\",\"label\":\"R\",\"type\":\"foundation.mechanical.rotational.rotational\"}],\"Right\":[{\"id\":\"C\",\"label\":\"C\",\"type\":\"foundation.mechanical.rotational.rotational\"},{\"id\":\"W\",\"label\":\"W\",\"type\":\"output\"}],\"Top\":[]}"
  PS-Simulink Converter : nesl_utility/PS-Simulink Converter  PhysicalDomain=network_engine_domain  SubClassName=ps_output  LeftPortType=input  RightPortType=output  PseudoPeriodic=off  Frequencies=[]  VectorFormat=inherit  Unit=rpm  AffineConversion=off
  R : PMIOPort  Side=Left
  w : Outport
  wires:
  PS-Simulink Converter/1 -> w/1
  connections:
  PS-Simulink Converter/LConn1 -- Motion Sensor/RConn2
  MRRef/LConn1 -- Motion Sensor/RConn1
  R/RConn1 -- Motion Sensor/LConn1

== system sm_wheel_loader_lib/CVT Power Split Hydromechanical/Sensor wP4c ==
  MRRef : fl_lib/Mechanical/Rotational Elements/Mechanical Rotational Reference
  Motion Sensor : fl_lib/Mechanical/Mechanical Sensors/Ideal Rotational Motion Sensor  reference=foundation.enum.MeasurementReference.difference  acceleration_port=false  velocity_port=true  position_port=false  wrap_angle=false  offset=0 rad
      settings: InternalSimscapePortConfiguration="{\"Bottom\":[],\"Left\":[{\"id\":\"R\",\"label\":\"R\",\"type\":\"foundation.mechanical.rotational.rotational\"}],\"Right\":[{\"id\":\"C\",\"label\":\"C\",\"type\":\"foundation.mechanical.rotational.rotational\"},{\"id\":\"W\",\"label\":\"W\",\"type\":\"output\"}],\"Top\":[]}"
  PS-Simulink Converter : nesl_utility/PS-Simulink Converter  PhysicalDomain=network_engine_domain  SubClassName=ps_output  LeftPortType=input  RightPortType=output  PseudoPeriodic=off  Frequencies=[]  VectorFormat=inherit  Unit=rpm  AffineConversion=off
  R : PMIOPort  Side=Left
  w : Outport
  wires:
  PS-Simulink Converter/1 -> w/1
  connections:
  PS-Simulink Converter/LConn1 -- Motion Sensor/RConn2
  MRRef/LConn1 -- Motion Sensor/RConn1
  R/RConn1 -- Motion Sensor/LConn1

== system sm_wheel_loader_lib/CVT Power Split Hydromechanical/Sensor wP4r ==
  MRRef : fl_lib/Mechanical/Rotational Elements/Mechanical Rotational Reference
  Motion Sensor : fl_lib/Mechanical/Mechanical Sensors/Ideal Rotational Motion Sensor  reference=foundation.enum.MeasurementReference.difference  acceleration_port=false  velocity_port=true  position_port=false  wrap_angle=false  offset=0 rad
      settings: InternalSimscapePortConfiguration="{\"Bottom\":[],\"Left\":[{\"id\":\"R\",\"label\":\"R\",\"type\":\"foundation.mechanical.rotational.rotational\"}],\"Right\":[{\"id\":\"C\",\"label\":\"C\",\"type\":\"foundation.mechanical.rotational.rotational\"},{\"id\":\"W\",\"label\":\"W\",\"type\":\"output\"}],\"Top\":[]}"
  PS-Simulink Converter : nesl_utility/PS-Simulink Converter  PhysicalDomain=network_engine_domain  SubClassName=ps_output  LeftPortType=input  RightPortType=output  PseudoPeriodic=off  Frequencies=[]  VectorFormat=inherit  Unit=rpm  AffineConversion=off
  R : PMIOPort  Side=Left
  w : Outport
  wires:
  PS-Simulink Converter/1 -> w/1
  connections:
  R/RConn1 -- Motion Sensor/LConn1
  MRRef/LConn1 -- Motion Sensor/RConn1
  PS-Simulink Converter/LConn1 -- Motion Sensor/RConn2

== system sm_wheel_loader_lib/CVT Power Split Hydromechanical/Sensor wP4s ==
  MRRef : fl_lib/Mechanical/Rotational Elements/Mechanical Rotational Reference
  Motion Sensor : fl_lib/Mechanical/Mechanical Sensors/Ideal Rotational Motion Sensor  reference=foundation.enum.MeasurementReference.difference  acceleration_port=false  velocity_port=true  position_port=false  wrap_angle=false  offset=0 rad
      settings: InternalSimscapePortConfiguration="{\"Bottom\":[],\"Left\":[{\"id\":\"R\",\"label\":\"R\",\"type\":\"foundation.mechanical.rotational.rotational\"}],\"Right\":[{\"id\":\"C\",\"label\":\"C\",\"type\":\"foundation.mechanical.rotational.rotational\"},{\"id\":\"W\",\"label\":\"W\",\"type\":\"output\"}],\"Top\":[]}"
  PS-Simulink Converter : nesl_utility/PS-Simulink Converter  PhysicalDomain=network_engine_domain  SubClassName=ps_output  LeftPortType=input  RightPortType=output  PseudoPeriodic=off  Frequencies=[]  VectorFormat=inherit  Unit=rpm  AffineConversion=off
  R : PMIOPort  Side=Left
  w : Outport
  wires:
  PS-Simulink Converter/1 -> w/1
  connections:
  PS-Simulink Converter/LConn1 -- Motion Sensor/RConn2
  MRRef/LConn1 -- Motion Sensor/RConn1
  R/RConn1 -- Motion Sensor/LConn1

== system sm_wheel_loader_lib/Controller/CVT Ratio Ctrl ==
  Ratio (-) : Inport
  CmdVehSpdDir : Inport  Port=2
  HRBCtrl (-) : Inport  Port=3
  MBCtrl (-) : Inport  Port=4
  Bus Creator : BusCreator  Inputs=12
  Clutch Truth Table : Stateflow chart  TreatAsAtomicUnit=on
  Filter : StateSpace  A=-200  C=200  D=0  InitialCondition=HMPST.Ctrl.Swash.XY_A(1,1)/200
  Range Calculation : Subsystem  mask{XY_I=HMPST.Ctrl.Swash.XY_I}
      mask prompts: XY_I "Range Separation Points"
  Saturation : Saturate  UpperLimit=HMPST.DesignReq.MaxCVTOutputSpeed/HMPST.Eng.wTarget  LowerLimit=0  ZeroCross=off
  Swash Ctrl : Lookup_n-D  NumberOfTableDimensions=1  BreakpointsForDimension1=HMPST.Ctrl.Swash.XY_A(:,2)  BeginIndexSearchUsingPreviousIndexResult=on  Table=HMPST.Ctrl.Swash.XY_A(:,1)  InternalRulePriority=Speed  RndMeth=Simplest
  Transfer Fcn : TransferFcn  Denominator=[0.1 1]
  CVT Ctrl : Outport
  wires:
  Ratio (-)/1 -> [ratio], Transfer Fcn/1
  Clutch Truth Table/1(K1Actv) -> Bus Creator/1  "K1"
  Clutch Truth Table/2(K2Actv) -> Bus Creator/2  "K2"
  Clutch Truth Table/3(K3Actv) -> Bus Creator/3  "K3"
  Clutch Truth Table/4(K4Actv) -> Bus Creator/4  "K4"
  Clutch Truth Table/5(KbActv) -> Bus Creator/5  "Kb"
  Clutch Truth Table/6(KvActv) -> Bus Creator/6  "Kv"
  Clutch Truth Table/7(KrActv) -> Bus Creator/7  "Kr"
  Bus Creator/1 -> CVT Ctrl/1  "Ctrl"
  Range Calculation/1(Range (-)) -> Clutch Truth Table/1(Range)
  Saturation/1 -> Swash Ctrl/1, Range Calculation/1(Ratio (-))
  Transfer Fcn/1 -> Saturation/1
  Filter/1 -> Bus Creator/12  "SwashCtrl"
  Swash Ctrl/1 -> Filter/1  "SwashCtrl"
  HRBCtrl (-)/1 -> Bus Creator/8  "HRBCtrl"
  MBCtrl (-)/1 -> Bus Creator/9  "MBCtrl"
  CmdVehSpdDir/1 -> Bus Creator/11, Clutch Truth Table/2(CmdVehSpdDir)  "CmdVehSpdDir"
  [ratio] -> Bus Creator/10  "ratio"

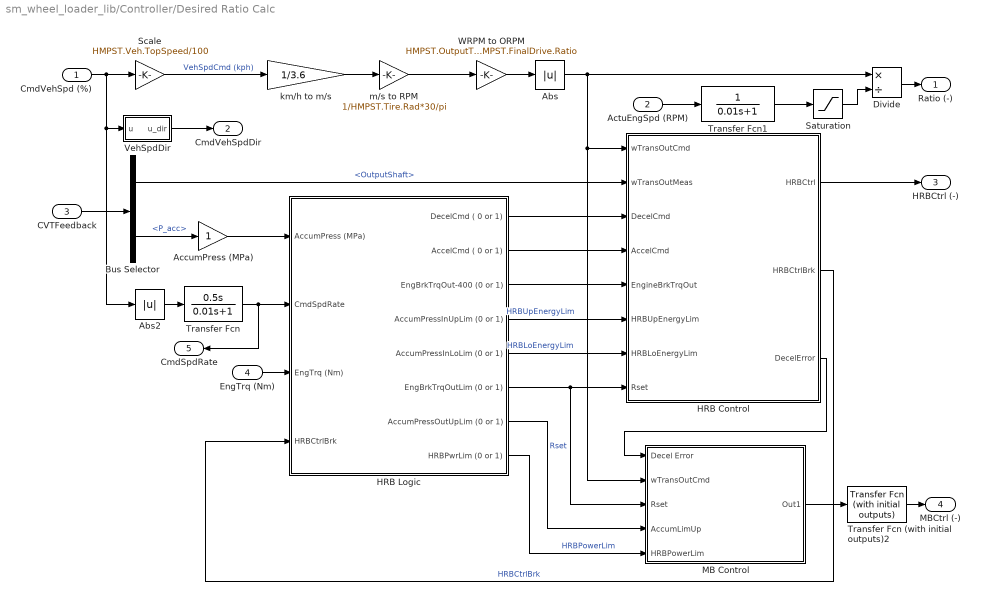
== system sm_wheel_loader_lib/Controller/Desired Ratio Calc ==
  CmdVehSpd (%) : Inport  SampleTime=HMPST.Simu.TimeStep
  ActuEngSpd (RPM) : Inport  Port=2
  CVTFeedback : Inport  Port=3
  EngTrq (Nm) : Inport  Port=4
  Abs : Abs  ZeroCross=off  SaturateOnIntegerOverflow=off
  Abs2 : Abs  ZeroCross=off  SaturateOnIntegerOverflow=off
  AccumPress (MPa) : Gain
  Bus Selector : BusSelector  OutputSignals=OutputShaft,P_acc
  Divide : Product  Inputs=*/
  HRB Control : Subsystem
  HRB Logic : Subsystem
  MB Control : Subsystem
  Saturation : Saturate  UpperLimit=2500  LowerLimit=0.5
  Scale : Gain  Gain=HMPST.Veh.TopSpeed/100
  Transfer Fcn : TransferFcn  Numerator=[0.5 0]  Denominator=[0.01 1]
  Transfer Fcn (with initial outputs)2 : simulink_extras/Additional Linear/Transfer Fcn (with initial outputs)  N=1  D=[0.05 1]  Y0=1  U0=1
  Transfer Fcn1 : TransferFcn  Denominator=[0.01 1]
  VehSpdDir : Subsystem
  WRPM to ORPM : Gain  Gain=HMPST.OutputTransferGearPair.Ratio*HMPST.Differential.Ratio*HMPST.FinalDrive.Ratio
  km/h to m/s : Gain  Gain=1/3.6
  m/s to RPM : Gain  Gain=1/HMPST.Tire.Rad*30/pi
  Ratio (-) : Outport
  CmdVehSpdDir : Outport  Port=2
  HRBCtrl (-) : Outport  Port=3
  MBCtrl (-) : Outport  Port=4
  CmdSpdRate : Outport  Port=5
  wires:
  MB Control/1(Out1) -> Transfer Fcn (with initial outputs)2/1
  HRB Logic/8(HRBPwrLim (0 or 1)) -> MB Control/5(HRBPowerLim)  "HRBPowerLim"
  HRB Logic/7(AccumPressOutUpLim (0 or 1)) -> MB Control/4(AccumLimUp)
  HRB Control/3(DecelError) -> MB Control/1(Decel Error)
  HRB Control/1(HRBCtrl) -> HRBCtrl (-)/1
  HRB Logic/3(EngBrkTrqOut-400 (0 or 1)) -> HRB Control/5(EngineBrkTrqOut)
  HRB Logic/2(AccelCmd ( 0 or 1)) -> HRB Control/4(AccelCmd)
  HRB Logic/5(AccumPressInLoLim (0 or 1)) -> HRB Control/7(HRBLoEnergyLim)  "HRBLoEnergyLim"
  HRB Logic/4(AccumPressInUpLim (0 or 1)) -> HRB Control/6(HRBUpEnergyLim)  "HRBUpEnergyLim"
  HRB Logic/1(DecelCmd ( 0 or 1)) -> HRB Control/3(DecelCmd)
  Divide/1 -> Ratio (-)/1
  ActuEngSpd (RPM)/1 -> Transfer Fcn1/1
  m/s to RPM/1 -> WRPM to ORPM/1
  km/h to m/s/1 -> m/s to RPM/1
  WRPM to ORPM/1 -> Abs/1
  CmdVehSpd (%)/1 -> Abs2/1, VehSpdDir/1(u), Scale/1
  Saturation/1 -> Divide/2
  Transfer Fcn1/1 -> Saturation/1
  Bus Selector/1 -> HRB Control/2(wTransOutMeas)  "<OutputShaft>"
  Transfer Fcn/1 -> HRB Logic/2(CmdSpdRate), CmdSpdRate/1
  CVTFeedback/1 -> Bus Selector/1
  HRB Logic/6(EngBrkTrqOutLim (0 or 1)) -> MB Control/3(Rset), HRB Control/8(Rset)  "Rset"
  Bus Selector/2 -> AccumPress (MPa)/1  "<P_acc>"
  EngTrq (Nm)/1 -> HRB Logic/3(EngTrq (Nm))
  AccumPress (MPa)/1 -> HRB Logic/1(AccumPress (MPa))
  VehSpdDir/1(u_dir) -> CmdVehSpdDir/1
  Scale/1 -> km/h to m/s/1  "VehSpdCmd (kph)"
  Abs2/1 -> Transfer Fcn/1
  Abs/1 -> Divide/1, MB Control/2(wTransOutCmd), HRB Control/1(wTransOutCmd)
  Transfer Fcn (with initial outputs)2/1 -> MBCtrl (-)/1
  HRB Control/2(HRBCtrlBrk) -> HRB Logic/4(HRBCtrlBrk)  "HRBCtrlBrk"

== system sm_wheel_loader_lib/Engine Droop/Speed Sensor ==
  MRRef : fl_lib/Mechanical/Rotational Elements/Mechanical Rotational Reference
  Motion Sensor : fl_lib/Mechanical/Mechanical Sensors/Ideal Rotational Motion Sensor  reference=foundation.enum.MeasurementReference.difference  acceleration_port=false  velocity_port=true  position_port=false  wrap_angle=false  offset=0 rad
      settings: InternalSimscapePortConfiguration="{\"Bottom\":[],\"Left\":[{\"id\":\"R\",\"label\":\"R\",\"type\":\"foundation.mechanical.rotational.rotational\"}],\"Right\":[{\"id\":\"C\",\"label\":\"C\",\"type\":\"foundation.mechanical.rotational.rotational\"},{\"id\":\"W\",\"label\":\"W\",\"type\":\"output\"}],\"Top\":[]}"
  Press A3 : nesl_utility/PS-Simulink Converter  PhysicalDomain=network_engine_domain  SubClassName=ps_output  LeftPortType=input  RightPortType=output  PseudoPeriodic=off  Frequencies=[]  VectorFormat=1-D array  Unit=rpm  AffineConversion=off
  Transfer Fcn : TransferFcn  Denominator=[0.1 1]
  R : PMIOPort  Side=Left
  rpm : Outport
  wires:
  Transfer Fcn/1 -> rpm/1
  Press A3/1 -> Transfer Fcn/1
  connections:
  R/RConn1 -- Motion Sensor/LConn1
  MRRef/LConn1 -- Motion Sensor/RConn1
  Motion Sensor/RConn2 -- Press A3/LConn1

== system sm_wheel_loader_lib/Engine Droop/Torque Sensor ==
  PS-Simulink Converter : nesl_utility/PS-Simulink Converter  PhysicalDomain=network_engine_domain  SubClassName=ps_output  LeftPortType=input  RightPortType=output  PseudoPeriodic=off  Frequencies=[]  VectorFormat=inherit  Unit=inherit  AffineConversion=off
  Torque Sensor : fl_lib/Mechanical/Mechanical Sensors/Ideal Torque Sensor
  R : PMIOPort  Side=Left
  C : PMIOPort  Port=2  Side=Right
  m : Outport
  wires:
  PS-Simulink Converter/1 -> m/1
  connections:
  PS-Simulink Converter/LConn1 -- Torque Sensor/RConn2
  Torque Sensor/LConn1 -- R/RConn1
  C/RConn1 -- Torque Sensor/RConn1

== system sm_wheel_loader_lib/Engine Generic/Speed Sensor ==
  Ideal Rotational Motion Sensor1 : fl_lib/Mechanical/Mechanical Sensors/Ideal Rotational Motion Sensor  reference=foundation.enum.MeasurementReference.difference  acceleration_port=false  velocity_port=true  position_port=false  wrap_angle=false  offset=0 rad
      settings: InternalSimscapePortConfiguration="{\"Bottom\":[],\"Left\":[{\"id\":\"R\",\"label\":\"R\",\"type\":\"foundation.mechanical.rotational.rotational\"}],\"Right\":[{\"id\":\"C\",\"label\":\"C\",\"type\":\"foundation.mechanical.rotational.rotational\"},{\"id\":\"W\",\"label\":\"W\",\"type\":\"output\"}],\"Top\":[]}"
  Mechanical Rotational Reference1 : fl_lib/Mechanical/Rotational Elements/Mechanical Rotational Reference
  Press A3 : nesl_utility/PS-Simulink Converter  PhysicalDomain=network_engine_domain  SubClassName=ps_output  LeftPortType=input  RightPortType=output  PseudoPeriodic=off  Frequencies=[]  VectorFormat=1-D array  Unit=rpm  AffineConversion=off
  Transfer Fcn : TransferFcn  Denominator=[0.1 1]
  R : PMIOPort  Side=Left
  w (rpm) : Outport
  wires:
  Transfer Fcn/1 -> w (rpm)/1
  Press A3/1 -> Transfer Fcn/1
  connections:
  R/RConn1 -- Ideal Rotational Motion Sensor1/LConn1
  Mechanical Rotational Reference1/LConn1 -- Ideal Rotational Motion Sensor1/RConn1
  Ideal Rotational Motion Sensor1/RConn2 -- Press A3/LConn1

== system sm_wheel_loader_lib/Engine Generic/Subsystem ==
  Ideal Torque Sensor : fl_lib/Mechanical/Mechanical Sensors/Ideal Torque Sensor
  PS-Simulink Converter : nesl_utility/PS-Simulink Converter  PhysicalDomain=network_engine_domain  SubClassName=ps_output  LeftPortType=input  RightPortType=output  PseudoPeriodic=off  Frequencies=[]  VectorFormat=inherit  Unit=inherit  AffineConversion=off
  R : PMIOPort  Side=Left
  C : PMIOPort  Port=2  Side=Right
  m : Outport
  wires:
  PS-Simulink Converter/1 -> m/1
  connections:
  PS-Simulink Converter/LConn1 -- Ideal Torque Sensor/RConn2
  Ideal Torque Sensor/LConn1 -- R/RConn1
  C/RConn1 -- Ideal Torque Sensor/RConn1

== system sm_wheel_loader_lib/Wheel Loader Vehicle/Actuators ==
  Cmd : Inport
  pwr : Inport  Port=2
  Hydraulic : Subsystem  VariantControl=Hydraulic  mask{popup_impl=Bucket}
      mask prompts: popup_impl "Implement"
      mask init:
      | if(strcmp(get_param(gcb,'popup_impl'),'Bucket'))
      |     set_param([gcb '/Implement'],'LabelModeActiveChoice','Bucket');
      | else
      |     set_param([gcb '/Implement'],'LabelModeActiveChoice','Grapple');
      | end
      mask TypeOptions popup_impl: Bucket | Grapple
      mask Display: image('sm_wheel_loader_actuators_hydraulic_IMAGE.png')
  Ideal : Subsystem  VariantControl=Ideal
      mask Display: image('sm_wheel_loader_actuators_ideal_IMAGE.png')
  LiftL : PMIOPort  Side=Right
  LiftR : PMIOPort  Port=2  Side=Right
  PTO : PMIOPort  Port=3  Side=Left
  RTilt : PMIOPort  Port=4  Side=Left
  Impl : PMIOPort  Port=5  Side=Right
  Steer : PMIOPort  Port=6  Side=Right
  SWhl : PMIOPort  Port=7  Side=Left
